simulink model "ModelSimulation_lab5"  (R2025b)
settings: Solver=VariableStepAuto  StartTime=0.0  StopTime=20  MaxStep=0.1  RelTol=1e-3
values from neighbouring files (symbols this model uses):
  A = [A1;A2;A3;A4;A5;A6;A7;A8;A9;A10;A11;A12;A13;A14;A15;A16;A17;A18;A19]    [lab5_2026.m]
  B = zeros(19,2)    [lab5_2026.m]
  CC = zeros(2,19)    [lab5_2026.m]
  D = zeros(2,2)    [lab5_2026.m]
  g = 9.8    [lab5_2026.m]
  U0 = TM0 * R / Kt    (= 1.3117040087)    [lab5_2026.m]
settings Model: Creator=yonmi  LastModifiedBy=yonmi
settings ModelReferenceCC: EnableRefExpFcnMdlSchedulingChecks=on
settings RTWCC: GPUComputeCapability=3.5

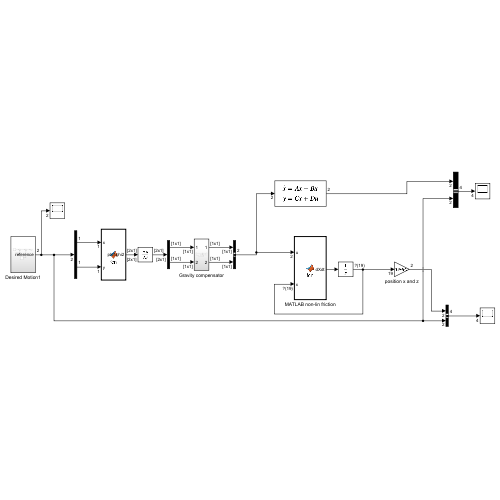
[thumbnail: Simulink's stored preview of the top-level diagram]
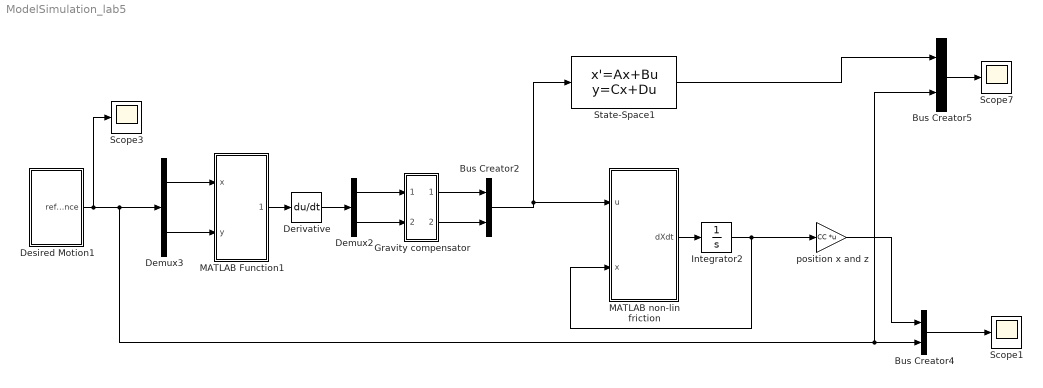
== system ModelSimulation_lab5 ==
  Bus Creator2 : BusCreator  Inputs=2
  Bus Creator4 : BusCreator  Inputs=2
  Bus Creator5 : BusCreator  Inputs=2
  Demux2 : Demux  Outputs=2
  Demux3 : Demux  Outputs=2
  Derivative : Derivative  CoefficientInTFapproximation=10
  Desired Motion1 : Subsystem
  Gravity compensator : Subsystem
  Integrator2 : Integrator  InitialCondition=[0 0 0 0 0 0 0 0 0 0 0 0 0 0 0 0 0 0 g]'
  MATLAB Function1 : MATLAB Function  TreatAsAtomicUnit=on
  MATLAB non-lin friction : MATLAB Function  TreatAsAtomicUnit=on
  Scope1 : Scope
      settings: ActiveDisplayYMinimum=-0.02861  ActiveDisplayYMaximum=0.02879  DataLoggingVariableName=ScopeData6  DataLoggingSaveFormat=Array
  Scope3 : Scope
      settings: ActiveDisplayYMinimum=-0.039163554454793768  ActiveDisplayYMaximum=0.036852670928329244  DataLoggingSaveFormat=Array
  Scope7 : Scope
      settings: ActiveDisplayYMinimum=-0.044708990791813938  ActiveDisplayYMaximum=0.037950661710412364  DataLoggingVariableName=ScopeData2
  State-Space1 : StateSpace  A=A  B=B  C=CC  D=D  InitialCondition=[0 0 0 0 0 0 0 0 0 0 0 0 0 0 0 0 0 0 g]'
  position x and z : Gain  Gain=CC  Multiplication=Matrix(K*u) (u vector)
  wires:
  position x and z/1 -> Bus Creator4/1
  Integrator2/1 -> position x and z/1, MATLAB non-lin friction/2(x)
  MATLAB non-lin friction/1(dXdt) -> Integrator2/1
  Bus Creator2/1 -> MATLAB non-lin friction/1(u), State-Space1/1
  Bus Creator4/1 -> Scope1/1
  Bus Creator5/1 -> Scope7/1
  State-Space1/1 -> Bus Creator5/1
  Demux3/1 -> MATLAB Function1/1(x)
  Demux3/2 -> MATLAB Function1/2(y)
  Desired Motion1/1(reference) -> Demux3/1, Bus Creator5/2, Bus Creator4/2, Scope3/1
  Derivative/1 -> Demux2/1
  MATLAB Function1/1(phi1phi2) -> Derivative/1
  Demux2/1 -> Gravity compensator/1(In1)
  Demux2/2 -> Gravity compensator/2(In2)
  Gravity compensator/1(Out1) -> Bus Creator2/1
  Gravity compensator/2(Out2) -> Bus Creator2/2

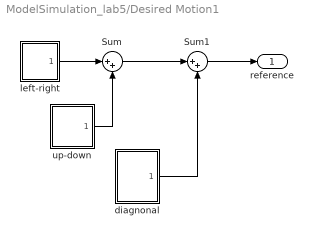
== system ModelSimulation_lab5/Desired Motion1 ==
  Sum : Sum  Inputs=|++
  Sum1 : Sum  Inputs=|++
  diagnonal : Subsystem
  left-right : Subsystem
  up-down : Subsystem
  reference : Outport
  wires:
  left-right/1(pxpy) -> Sum/1
  Sum/1 -> Sum1/1
  diagnonal/1(pxpy2) -> Sum1/2
  up-down/1(pxpy1) -> Sum/2
  Sum1/1 -> reference/1

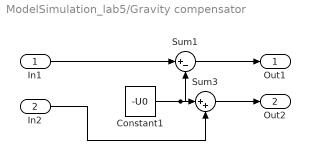
== system ModelSimulation_lab5/Gravity compensator ==
  In1 : Inport
  In2 : Inport  Port=2
  Constant1 : Constant  Value=-U0
  Sum1 : Sum  Inputs=|+-
  Sum3 : Sum  Inputs=|++
  Out1 : Outport
  Out2 : Outport  Port=2
  wires:
  Constant1/1 -> Sum3/1, Sum1/2
  Sum1/1 -> Out1/1
  In1/1 -> Sum1/1
  In2/1 -> Sum3/2
  Sum3/1 -> Out2/1

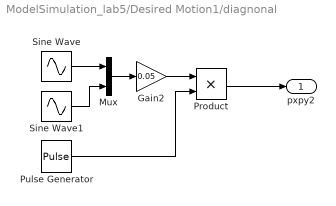
== system ModelSimulation_lab5/Desired Motion1/diagnonal ==
  Gain2 : Gain  Gain=0.05
  Mux : Mux  Inputs=2
  Product : Product
  Pulse Generator : DiscretePulseGenerator  PulseType=Time based  Amplitude=0.5  Period=15  PulseWidth=16.667  PhaseDelay=5
  Sine Wave : Sin  Amplitude=0.5  Frequency=2*pi/2.5  SampleTime=0
  Sine Wave1 : Sin  Amplitude=0.5  Frequency=2*pi/2.5  SampleTime=0
  pxpy2 : Outport  VectorParamsAs1DForOutWhenUnconnected=off
  wires:
  Product/1 -> pxpy2/1
  Mux/1 -> Gain2/1
  Pulse Generator/1 -> Product/2
  Sine Wave/1 -> Mux/1
  Sine Wave1/1 -> Mux/2
  Gain2/1 -> Product/1

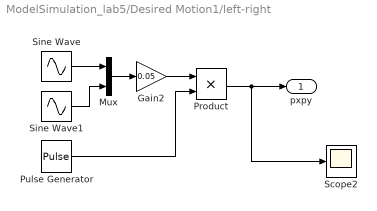
== system ModelSimulation_lab5/Desired Motion1/left-right ==
  Gain2 : Gain  Gain=0.05
  Mux : Mux  Inputs=2
  Product : Product
  Pulse Generator : DiscretePulseGenerator  PulseType=Time based  Amplitude=0.5  Period=15  PulseWidth=16.667
  Scope2 : Scope
      settings: ActiveDisplayYMinimum=-0.0625  ActiveDisplayYMaximum=0.0625  DataLoggingVariableName=ScopeData2  DataLoggingSaveFormat=Array
  Sine Wave : Sin  Amplitude=0.5  Frequency=2*pi/2.5  SampleTime=0
  Sine Wave1 : Sin  Amplitude=-1*0  Frequency=2*pi/2.5  SampleTime=0
  pxpy : Outport  VectorParamsAs1DForOutWhenUnconnected=off
  wires:
  Product/1 -> pxpy/1, Scope2/1
  Pulse Generator/1 -> Product/2
  Mux/1 -> Gain2/1
  Sine Wave1/1 -> Mux/2
  Sine Wave/1 -> Mux/1
  Gain2/1 -> Product/1

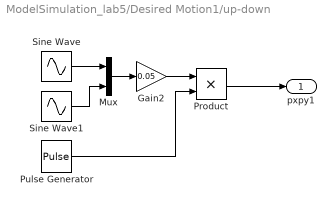
== system ModelSimulation_lab5/Desired Motion1/up-down ==
  Gain2 : Gain  Gain=0.05
  Mux : Mux  Inputs=2
  Product : Product
  Pulse Generator : DiscretePulseGenerator  PulseType=Time based  Amplitude=0.5  Period=15  PulseWidth=16.667  PhaseDelay=2.5
  Sine Wave : Sin  Amplitude=1*0  Frequency=2*pi/2.5  SampleTime=0
  Sine Wave1 : Sin  Amplitude=0.5  Frequency=2*pi/2.5  SampleTime=0
  pxpy1 : Outport  VectorParamsAs1DForOutWhenUnconnected=off
  wires:
  Sine Wave1/1 -> Mux/2
  Product/1 -> pxpy1/1
  Gain2/1 -> Product/1
  Mux/1 -> Gain2/1
  Pulse Generator/1 -> Product/2
  Sine Wave/1 -> Mux/1

== matlab function ModelSimulation_lab5/MATLAB Function1 ==
  data: x input; y input; phi1phi2 output
function phi1phi2= fcn(x,y)
%%%parameters

phi1phi2=90*inv([1 1;-1 1])*[x; y];

end

== matlab function ModelSimulation_lab5/MATLAB non-lin friction ==
  data: u input; x input; dXdt output
function dXdt = fcn(u,x)
%x is the state here
%%%parameters
r=0.0194;
rp=0.0194;
R0=0.0194;
M=0.001;
m=0.001;
mp=0.001;
Mb=0.446;
Mc=4.07; 
g=9.8;
J=5.6e-5;
J1=5.6e-5;
J2=5.6e-5;
J3=5.6e-5;
J4=5.6e-5;
J5=5.6e-5; 

Bc=23.2224; 
Bc=40;
Bb=46.4449;
B1=0.0021;
B2=0.0021;
B3=0.0021;
B4=0.0021;
B5=0.0021;
B0=0.0021;

% Fc=0.20;
% Fs=0.001;
% Ft=100000;
% N=1000;


Fc=0.16;
Fs=.13;
Ft=100000;
N=1000;

Kt=0.023;
Ke=0.023;
R=0.71;
k1=17810;
k2=17810;
k5=17810;
k6=17810;
k3=12565;
k4=12565;
k7=25013;
k8=25013;
U=Mb + Mc + 4*m + mp;
E=Mb + mp;

%%%%%%%%%%%%%%%%%%%%%%%%%%%%%%%%%%%%%%%%
dx1dt=x(2);


% syms x z ha hb h1 h2 h3 h4 h5% q
% syms dx dz dha dhb dh1 dh2 dh3 dh4 dh5 %first order derivertive
% syms dot2x dot2z dot2ha dot2hb dot2h1 dot2h2 dot2h3 dot2h4 dot2h5 %second order derivertive

%dx2dt:GET IT FROM YOUR SYBOLIC COMPUTATION FILE,  AND REPRESENT IT BY X
%STATE
dx2dt=

dx3dt=x(4);
%Compplete the rest yourself

dx19dt=0;

dXdt=[dx1dt dx2dt dx3dt dx4dt dx5dt dx6dt dx7dt dx8dt dx9dt dx10dt dx11dt dx12dt dx13dt dx14dt dx15dt dx16dt dx17dt dx18dt dx19dt]';
end
